simulink model "withoutDOS"  (R2018b)
settings: Solver=VariableStepAuto  StartTime=0.0  StopTime=30  RelTol=1e-3
settings Model: Creator=lenovo  LastModifiedBy=lenovo

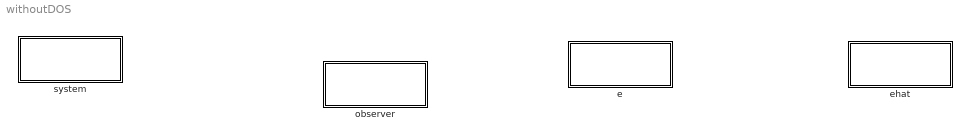
== system withoutDOS ==
  e : Subsystem
  ehat : Subsystem
  observer : Subsystem
  system : Subsystem

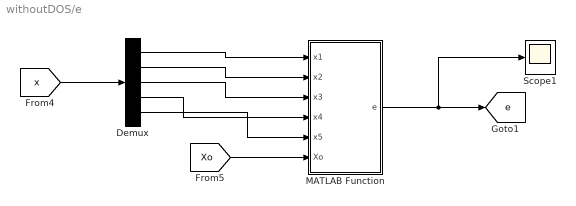
== system withoutDOS/e ==
  Demux : Demux  Outputs=5
  MATLAB Function : MATLAB Function  TreatAsAtomicUnit=on
  Scope1 : Scope
  tag scope: e=global
  wires:
  MATLAB Function/1(e) -> Scope1/1, [e]
  Demux/2 -> MATLAB Function/2(x2)
  Demux/1 -> MATLAB Function/1(x1)
  Demux/5 -> MATLAB Function/5(x5)
  [x] -> Demux/1
  Demux/4 -> MATLAB Function/4(x4)
  [Xo] -> MATLAB Function/6(Xo)
  Demux/3 -> MATLAB Function/3(x3)

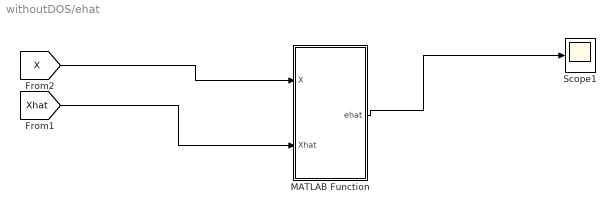
== system withoutDOS/ehat ==
  MATLAB Function : MATLAB Function  TreatAsAtomicUnit=on
  Scope1 : Scope
  wires:
  MATLAB Function/1(ehat) -> Scope1/1
  [X] -> MATLAB Function/1(X)
  [Xhat] -> MATLAB Function/2(Xhat)

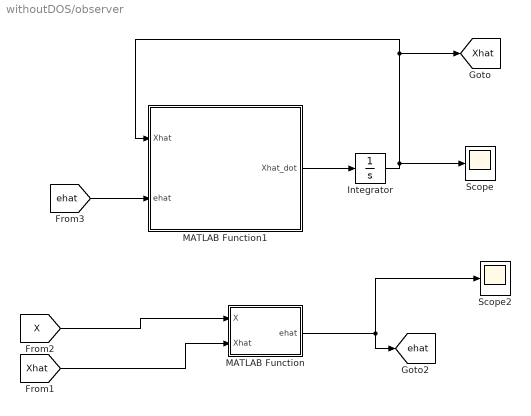
== system withoutDOS/observer ==
  Integrator : Integrator  InitialCondition=[-0.5;-1;-1.5;-2;-2.5;-3;-3.5;-4;-4.5;-5;-5.5;-6;0.5;1;1.5;2;2.5;3;3.5;4;4.5;5;5.5;6]
  MATLAB Function : MATLAB Function  TreatAsAtomicUnit=on
  MATLAB Function1 : MATLAB Function  TreatAsAtomicUnit=on
  Scope : Scope
  Scope2 : Scope
  tag scope: Xhat=global, ehat=global
  wires:
  MATLAB Function1/1(Xhat_dot) -> Integrator/1
  Integrator/1 -> Scope/1, [Xhat], MATLAB Function1/1(Xhat)
  [ehat] -> MATLAB Function1/2(ehat)
  MATLAB Function/1(ehat) -> [ehat], Scope2/1
  [X] -> MATLAB Function/1(X)
  [Xhat] -> MATLAB Function/2(Xhat)

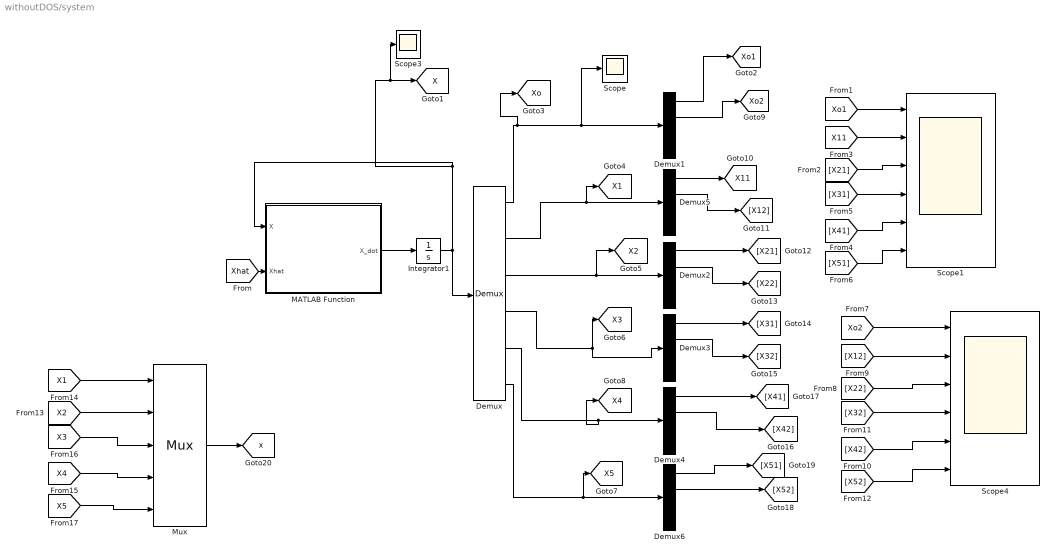
== system withoutDOS/system ==
  Demux : Demux  Outputs=6
  Demux{1..6} (6 alike) : Demux
  Integrator1 : Integrator  InitialCondition=[-0.5;-1;-1.5;-2;-2.5;-3;-3.5;-4;-4.5;-5;-5.5;-6;0.5;1;1.5;2;2.5;3;3.5;4;4.5;5;5.5;6]
  MATLAB Function : MATLAB Function  TreatAsAtomicUnit=on
  Mux : Mux  Inputs=5
  Scope : Scope
  Scope1 : Scope  NumInputPorts=6
  Scope3 : Scope
  Scope4 : Scope  NumInputPorts=6
  tag scope: X11=global, X1=global, X2=global, X3=global, X4=global, X5=global, X=global, Xo1=global, Xo2=global, Xo=global, x=global
  wires:
  Demux/2 -> [X1], Demux5/1
  Demux/3 -> [X2], Demux2/1
  Demux/1 -> [Xo], Scope/1, Demux1/1
  Demux/4 -> [X3], Demux3/1
  Demux/6 -> [X5], Demux6/1
  Demux/5 -> [X4], Demux4/1
  [Xhat] -> MATLAB Function/2(Xhat)
  MATLAB Function/1(X_dot) -> Integrator1/1
  Integrator1/1 -> MATLAB Function/1(X), Scope3/1, [X], Demux/1
  Demux1/1 -> [Xo1]
  Demux1/2 -> [Xo2]
  Demux5/1 -> [X11]
  Demux5/2 -> [X12]
  Demux2/1 -> [X21]
  Demux2/2 -> [X22]
  Demux3/1 -> [X31]
  Demux3/2 -> [X32]
  Demux4/1 -> [X41]
  Demux4/2 -> [X42]
  Demux6/1 -> [X51]
  Demux6/2 -> [X52]
  [Xo1] -> Scope1/1
  [X11] -> Scope1/2
  [X21] -> Scope1/3
  [X31] -> Scope1/4
  [X41] -> Scope1/5
  [X51] -> Scope1/6
  [X52] -> Scope4/6
  [X22] -> Scope4/3
  [X32] -> Scope4/4
  [X12] -> Scope4/2
  [X42] -> Scope4/5
  [Xo2] -> Scope4/1
  [X1] -> Mux/1
  [X2] -> Mux/2
  [X3] -> Mux/3
  [X4] -> Mux/4
  [X5] -> Mux/5
  Mux/1 -> [x]

== matlab function withoutDOS/observer/MATLAB Function1 ==
  data: Xhat input; Xhat_dot output; ehat input
function Xhat_dot = X(Xhat,ehat)
A=[0 1 0 0;-48.6 -1.26 48.6 0;0 0 0 10; 1.95 0 -1.95 0];
B=[0;21.6;0;0];
C=[1 0 1 -1;0 1 0 0];
c=2;
teta=5;
H=[3.0849 0.6931;2.4258 34.9384;7.0235 3.5334;.54 1.8007];


N=6;

L=[0 0 0 0 0 0;-1 2 0 0 0 -1;-1 -1 2 0 0 0;0 -1 0 1 0 0;0 0 -1 0 1 0;0 0 -1 -1 -1 3];
K=[79.1094 5.2218 -29.6598 163.9093];




A0=kron(eye(N),A);
z1=kron(L,B*K);
z2=kron(L,H*C);
 

Xhat_dot= (A0-c*z1)*Xhat+teta*(z2*ehat);

== matlab function withoutDOS/system/MATLAB Function ==
  data: X input; X_dot output; Xhat input
function X_dot = X(X,Xhat)
A=[0 1 0 0;-48.6 -1.26 48.6 0;0 0 0 10; 1.95 0 -1.95 0];
B=[0;21.6;0;0];
C=[1 0 1 -1;0 1 0 0];
c=2;

N=6;

L=[0 0 0 0 0 0;-1 2 0 0 0 -1;-1 -1 2 0 0 0;0 -1 0 1 0 0;0 0 -1 0 1 0;0 0 -1 -1 -1 3];
K=[79.1094 5.2218 -29.6598 163.9093];



A0=kron(eye(N),A);
z1=kron(L,B*K);
 


X_dot= A0*X-c*(z1*Xhat);

== matlab function withoutDOS/e/MATLAB Function ==
  data: x1 input; x2 input; x3 input; x4 input; x5 input; e output; Xo input
function e = fcn(x1,x2,x3,x4,x5,Xo)

e =0.2* norm(x1-Xo+x2-Xo+x3-Xo+x4-Xo+x5-Xo);

== matlab function withoutDOS/ehat/MATLAB Function ==
  data: X input; Xhat input; ehat output
function ehat = fcn(X,Xhat)

ehat = norm(X-Xhat);

== matlab function withoutDOS/observer/MATLAB Function ==
  data: X input; ehat output; Xhat input
function ehat = fcn(X,Xhat)

ehat =( X-Xhat);
